simulink model "SZ09_BC"  (R2026a)
settings: Solver=VariableStepAuto  StopTime=2  MaxStep=1e-3
libraries: simulink_extras x1
settings Model: Creator=Szalay  LastModifiedBy=Szalay

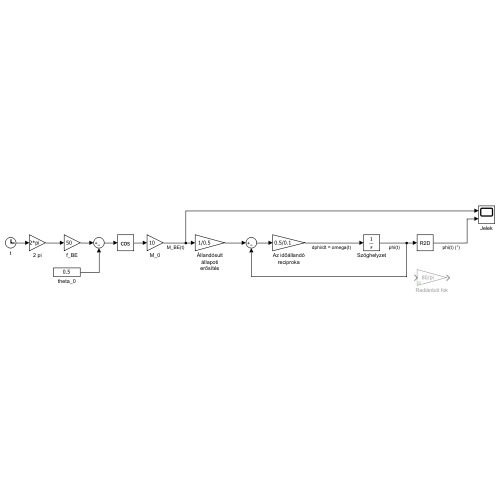
[thumbnail: Simulink's stored preview of the top-level diagram]
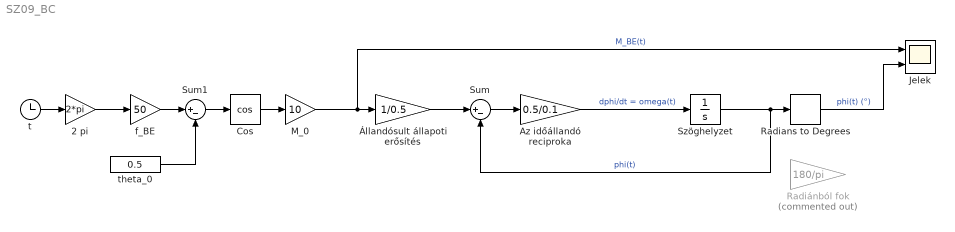
== system SZ09_BC ==
  2 pi : Gain  Gain=2*pi
  Az időállandó reciproka : Gain  Gain=0.5/0.1
  Cos : Trigonometry  Operator=cos
  Jelek : Scope  NumInputPorts=2
      settings: ActiveDisplayYMinimum=-27.215203699691994  ActiveDisplayYMaximum=64.493019978890686
  M_0 : Gain  Gain=10
  Radians to Degrees : simulink_extras/Transformations/Radians to Degrees
  Radiánból fok : Gain  Commented=on  Gain=180/pi
  Sum : Sum  Inputs=|+-
  Sum1 : Sum  Inputs=|+-
  Szöghelyzet : Integrator  InitialCondition=deg2rad(30)
  f_BE : Gain  Gain=50
  t : Clock
  theta_0 : Constant  Value=0.5
  Állandósult állapoti erősítés : Gain  Gain=1/0.5
  wires:
  Az időállandó reciproka/1 -> Szöghelyzet/1  "dphi/dt = omega(t)"
  Szöghelyzet/1 -> Radians to Degrees/1, Sum/2  "phi(t)"
  Sum/1 -> Az időállandó reciproka/1
  Állandósult állapoti erősítés/1 -> Sum/1
  M_0/1 -> Jelek/1, Állandósult állapoti erősítés/1  "M_BE(t)"
  t/1 -> 2 pi/1
  2 pi/1 -> f_BE/1
  f_BE/1 -> Sum1/1
  theta_0/1 -> Sum1/2
  Sum1/1 -> Cos/1
  Cos/1 -> M_0/1
  Radians to Degrees/1 -> Jelek/2  "phi(t) (°)"
